simulink model "transmitDSSS"  (R2021b)
settings: Solver=VariableStepAuto  StartTime=0.0  StopTime=10  RelTol=1e-3
InitFcn:
  | Tb = 1/1000;
  | Tc = 1/8000;
  | fs = 64e3;
  | Ts = 1/fs;
undefined symbols (not defined in the file or in its folder): designMultirateFIR, Fs, ip, usb
libraries: plutoradiolib x2, commsync2 x2, commfilt2 x2, dspsrcs4 x2, commdigbbndpm3 x1, dspmlti4 x1
settings Model: Creator=prust  LastModifiedBy=mhmma
settings SolverCC: AlgebraicLoopSolver=TrustRegion
settings DataIOCC: ReturnWorkspaceOutputs=off
settings DebuggingCC: SFMachineParentedDataDiag=warning  ArithmeticOperatorsInVariantConditions=warning
settings SFSimCC: SimUseLocalCustomCode=off  CustomCodeUndefinedFunction=UseInterfaceOnly
settings RTWCC: RTWUseLocalCustomCode=off
settings CodeAppCC: StateflowObjectComments=on

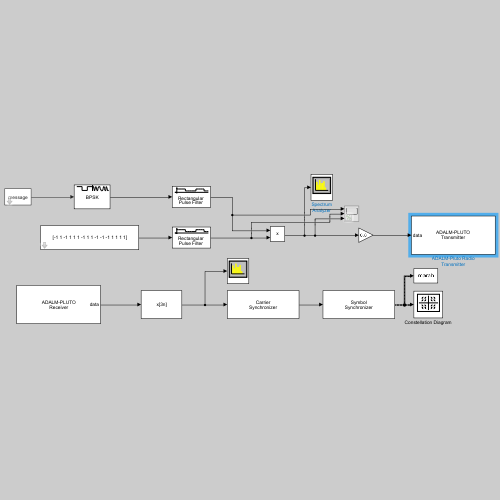
[thumbnail: Simulink's stored preview of the top-level diagram]
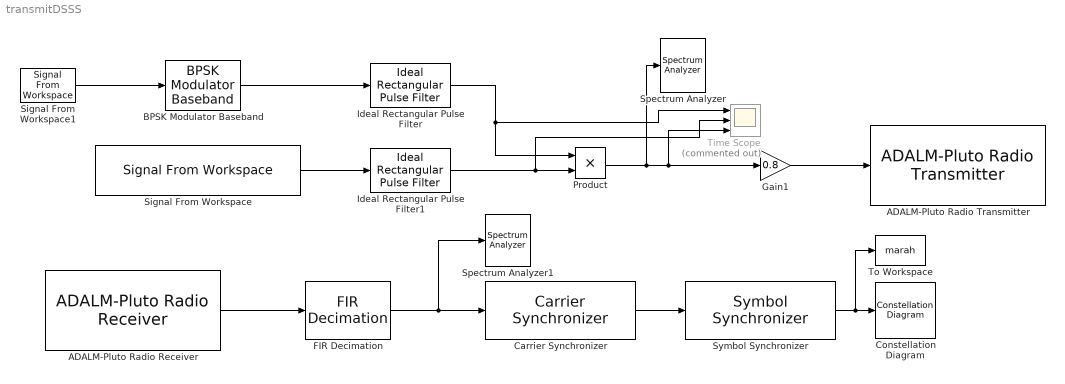
== system transmitDSSS ==
  ADALM-Pluto Radio Receiver : plutoradiolib/ADALM-Pluto Radio Receiver  RadioID=usb:0  uri=ip:10.0.0.200  CenterFrequencySource=Dialog  CenterFrequency=905e6  GainSource=AGC Slow Attack  GainSourceBlock=AGC Slow Attack  Gain=40  ChannelMapping=1  BasebandSampleRate=240e3  OutputDataType=single  SamplesPerFrame=120000  OverflowOutputPort=off  EnableBurstMode=off  NumFramesInBurst=1  ShowAdvancedProperties=off  UseCustomFilter=off  filtPathRates=[737280000 11520000 3840000 1920000 960000 240000]  filtCoefficients=[-192 82 85 -215 228 -102 -110 290 -318 145 160 -426 471 -215 -238 633 -697 318 349 -923 1009 -457 -498 1309 -1423 640 693 -1812 1959 -876 -945 2458 -2647 1180 1268 -3290 3534 -1572 -1688 4375 -4698 2091 2247 -5836 6284 -2807 -3031 7918 -8588 3870 4225 -11182 12324 -5662 -6330 17255 -19735 9507 11312 -33568 43355 -25227 -42139 305542 305542 -42139 -25227 43355 -33568 11312 9507 -19735 17255 -6330 -5662 12324 -11182 4225 3870 -8588 7918 -3031 -2807 6284 -5836 2247 2091 -4698 4375 -1688 -1572 3534 -3290 1268 1180 -2647 2458 -945 -876 1959 -1812 693 640 -1423 1309 -498 -457 1009 -923 349 318 -697 633 -238 -215 471 -426 160 145 -318 290 -110 -102 228 -215 85 82 -192]  filtCoefficientSize=128  filtDecimInterpFactor=4  filtGain=-12  filtRFBandwidth=18000000  filterConfigStruct=struct()  EnableQuadratureCorrection=on  EnableRFDCCorrection=on  EnableBasebandDCCorrection=on  FrequencyCorrection=0  OverrideSampleTime=off  SampleTime=0.02  DataTimeout=Inf  ENSMPinControlMode=None  BISTLoopbackMode=Disabled  BISTToneInject=Disabled  BISTSignalGen=PRBS  BISTToneFreq=Fs/32  BISTToneLevel=0
      settings: SourceProductBaseCode=PLUTO
  ADALM-Pluto Radio Transmitter : plutoradiolib/ADALM-Pluto Radio Transmitter  RadioID=usb:0  uri=ip:10.0.0.200  CenterFrequencySource=Dialog  CenterFrequency=905e6  GainSource=Dialog  Gain=-40  ChannelMapping=1  BasebandSampleRate=240e3  UnderflowOutputPort=off  ShowAdvancedProperties=off  UseCustomFilter=off  filtPathRates=[737280000 11520000 3840000 1920000 960000 240000]  filtCoefficients=[-192 82 85 -215 228 -102 -110 290 -318 145 160 -426 471 -215 -238 633 -697 318 349 -923 1009 -457 -498 1309 -1423 640 693 -1812 1959 -876 -945 2458 -2647 1180 1268 -3290 3534 -1572 -1688 4375 -4698 2091 2247 -5836 6284 -2807 -3031 7918 -8588 3870 4225 -11182 12324 -5662 -6330 17255 -19735 9507 11312 -33568 43355 -25227 -42139 305542 305542 -42139 -25227 43355 -33568 11312 9507 -19735 17255 -6330 -5662 12324 -11182 4225 3870 -8588 7918 -3031 -2807 6284 -5836 2247 2091 -4698 4375 -1688 -1572 3534 -3290 1268 1180 -2647 2458 -945 -876 1959 -1812 693 640 -1423 1309 -498 -457 1009 -923 349 318 -697 633 -238 -215 471 -426 160 145 -318 290 -110 -102 228 -215 85 82 -192]  filtCoefficientSize=128  filtDecimInterpFactor=4  filtGain=-12  filtRFBandwidth=18000000  filterConfigStruct=struct()  DataSourceSelect=Input Port  DDSTone1Freq=5e3  DDSTone2Freq=10e3  DDSTone1Scale=0.5  DDSTone2Scale=0.25  DataTimeout=Inf  FrequencyCorrection=0  ENSMPinControlMode=None  BISTLoopbackMode=Disabled  BISTToneInject=Disabled  BISTSignalGen=PRBS  BISTToneFreq=Fs/32  BISTToneLevel=0
      settings: SourceProductBaseCode=PLUTO
  BPSK Modulator Baseband : commdigbbndpm3/BPSK Modulator Baseband  Ph=0  outDtype=double  outWordLen=16  outUDDataType=sfix(16)  outFracLenMode=Best precision  outFracLen=15  outDataTypeStr=double  outLastDataTypeStr=double
  Carrier Synchronizer : commsync2/Carrier Synchronizer  Modulation=BPSK  ModulationPhaseOffset=Auto  CustomPhaseOffset=0  SamplesPerSymbol=10  DampingFactor=0.707  NormalizedLoopBandwidth=0.01  EstimatedPhaseErrorOutputPort=off  SimulateUsing=Code generation
  Constellation Diagram : ConstellationDiagram
  FIR Decimation : dspmlti4/FIR Decimation  FilterSource=Auto  h=designMultirateFIR(1,2)  D=3  filtStruct=Direct form  FilterObject=FDECIM  InputProcessing=Columns as channels (frame based)  framing=Enforce single-rate processing  inputOffset=0  outputBufInitCond=0  roundingMode=Floor  overflowMode=off  firstCoeffDataTypeStr=Inherit: Same word length as input  firstCoeffMin=[]  firstCoeffMax=[]  firstCoeffLastDataTypeStr=Inherit: Same word length as input  outputDataTypeStr=Inherit: Same as accumulator  outputMin=[]  outputMax=[]  outputLastDataTypeStr=Inherit: Same as accumulator
  Gain1 : Gain  Gain=0.8
  Ideal Rectangular Pulse Filter : commfilt2/Ideal Rectangular Pulse Filter  pulseLen=240  pulseDelay=0  InputProcessing=Columns as channels (frame based)  RateOptions=Allow multirate processing  sampMode=Mute  normCheck=off  normMode=Sum of samples  filterGain=1  saveAsFlag=0  roundingMode=Floor  overflowMode=off  firstCoeffDataTypeStr=Inherit: Same word length as input  firstCoeffMin=[]  firstCoeffMax=[]  firstCoeffLastDataTypeStr=Inherit: Same word length as input  outputDataTypeStr=Inherit: Same as accumulator  outputMin=[]  outputMax=[]  outputLastDataTypeStr=Inherit: Same as accumulator
      settings: SourceProductBaseCode=CM
  Ideal Rectangular Pulse Filter1 : commfilt2/Ideal Rectangular Pulse Filter  pulseLen=30  pulseDelay=0  InputProcessing=Columns as channels (frame based)  RateOptions=Allow multirate processing  sampMode=Mute  normCheck=off  normMode=Sum of samples  filterGain=1  saveAsFlag=0  roundingMode=Floor  overflowMode=off  firstCoeffDataTypeStr=Inherit: Same word length as input  firstCoeffMin=[]  firstCoeffMax=[]  firstCoeffLastDataTypeStr=Inherit: Same word length as input  outputDataTypeStr=Inherit: Same as accumulator  outputMin=[]  outputMax=[]  outputLastDataTypeStr=Inherit: Same as accumulator
      settings: SourceProductBaseCode=CM
  Product : Product
  Signal From Workspace : dspsrcs4/Signal From Workspace  X=[-1 1 -1 1 1 1 -1 1 1 -1 -1 -1 1 1 1 1]  Ts=Tc  nsamps=1600  OutputAfterFinalValue=Cyclic repetition  ignoreOrWarnInputAndFrameLengths=off  OutputFrames=off
  Signal From Workspace1 : dspsrcs4/Signal From Workspace  X=message  Ts=Tb  nsamps=1600  OutputAfterFinalValue=Cyclic repetition  ignoreOrWarnInputAndFrameLengths=off  OutputFrames=off
  Spectrum Analyzer : SpectrumAnalyzer
  Spectrum Analyzer1 : SpectrumAnalyzer
  Symbol Synchronizer : commsync2/Symbol Synchronizer  Modulation=PAM/PSK/QAM  TimingErrorDetector=Zero-Crossing (decision-directed)  SamplesPerSymbol=10  DampingFactor=1  NormalizedLoopBandwidth=0.01  DetectorGain=2.7  TimingErrorOutputPort=off  SimulateUsing=Code generation
      settings: SourceProductBaseCode=CM
  Time Scope : Scope  Commented=on  NumInputPorts=3
  To Workspace : ToWorkspace  VariableName=marah  SaveFormat=Structure  SampleTime=-1
      settings: MaxDataPoints=4000  Save2DSignal=2-D array (concatenate along first dimension)
  wires:
  Carrier Synchronizer/1 -> Symbol Synchronizer/1
  ADALM-Pluto Radio Receiver/1 -> FIR Decimation/1
  Signal From Workspace/1 -> Ideal Rectangular Pulse Filter1/1
  FIR Decimation/1 -> Spectrum Analyzer1/1, Carrier Synchronizer/1
  Symbol Synchronizer/1 -> To Workspace/1, Constellation Diagram/1
  Product/1 -> Spectrum Analyzer/1, Time Scope/3, Gain1/1
  Gain1/1 -> ADALM-Pluto Radio Transmitter/1
  BPSK Modulator Baseband/1 -> Ideal Rectangular Pulse Filter/1
  Signal From Workspace1/1 -> BPSK Modulator Baseband/1
  Ideal Rectangular Pulse Filter1/1 -> Time Scope/2, Product/2
  Ideal Rectangular Pulse Filter/1 -> Time Scope/1, Product/1
